simulink model "UR5e_Unreal_Checkpoint"  (R2025b)
settings: Solver=FixedStepDiscrete  StartTime=0.0  StopTime=stopTimeUE  FixedStep=0.02  RelTol=1e-3
values from neighbouring files (symbols this model uses):
  qUE = qMotion(1,:)    [UR5e_Prepare_Project.m]    (also in UR5e_UE_Scene.m)
undefined symbols (not defined in the file or in its folder): Actor, UR5e_Glue_Bead
libraries: sim3dlib x2, robotsim3dlib x1
settings Model: Creator=Lenovo  LastModifiedBy=Lenovo

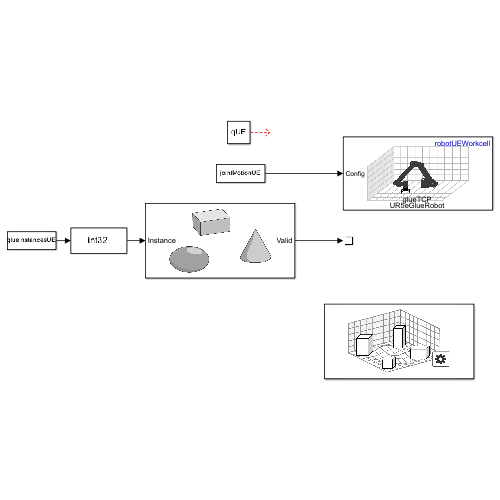
[thumbnail: Simulink's stored preview of the top-level diagram]
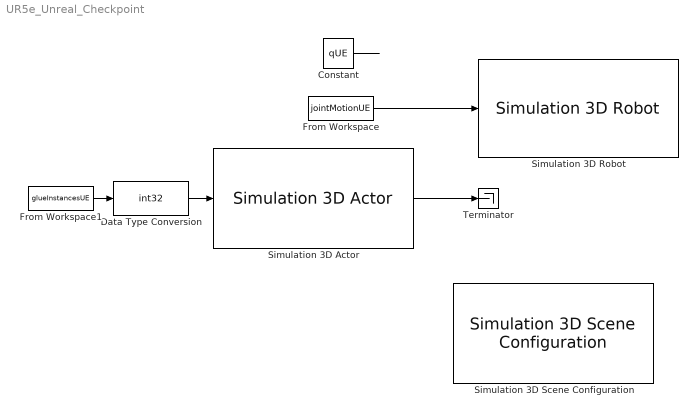
== system UR5e_Unreal_Checkpoint ==
  Constant : Constant  Value=qUE
  Data Type Conversion : DataTypeConversion  OutDataTypeStr=int32  SaturateOnIntegerOverflow=off  RndMeth=Floor
  From Workspace : FromWorkspace  VariableName=jointMotionUE  SampleTime=0.02  OutputAfterFinalValue=Holding final value
  From Workspace1 : FromWorkspace  VariableName=glueInstancesUE  SampleTime=0.02  Interpolate=off  OutputAfterFinalValue=Holding final value
  Simulation 3D Actor : sim3dlib/Simulation 3D Actor  Priority=-1  ActorName=GlueBead  ParentName=Scene Origin  Operation=Create at step  InitScriptText=UR5e_Glue_Bead('create', Actor);  SampleTime=-1  Translation=[0 0 0]  Rotation=[0 0 0]  Scale=[1 1 1]  aMode=5  ActorTag=Sim3dActor1  ActorType=Sim3dActor  ID=1
  Simulation 3D Robot : robotsim3dlib/Simulation 3D Robot  actorInputType=RigidBodyTree Object  RigidBodyTree=robotUEWorkcell  ActorName=UR5eGlueRobot  existActorChekBox=off  initialTrans=[0 0 0]  initialRot=[0 0 0]  initialConfig=qUE  EndEffector=glueTCP  eeOffsetInpChekBox=off  eeTargetTrans=[0 0 0]  eeTargetRot=[0 0 0]  enableRegionGraspChekBox=off  regionGraspInpChekBox=off  eeTargTransDiff=[0.2 0.2 0.2]  eeTargRotDiff=[0 0 0]  enableVisualVisualization=on  enableCollisionVisualization=off  collisionGeomColor=[0 1 0]  collisionGeomTransp=0.1  inpConfEnbVal=on  inpGraspEnbVal=off  inpTransEnbVal=off  outConfEnbVal=off  outGraspEnbVal=off  outTransEnbVal=off  SampleTime=0.02  ActorType=SimulinkVehicle  ID=C  aMode=6  ActorTag=UR5eGlueRobot  Mesh=RigidBodyTree
  Simulation 3D Scene Configuration : sim3dlib/Simulation 3D Scene Configuration  Priority=0  ProjectFormat=Default Scenes  SceneDesc=Empty scene  ProjectName=C:\Program Files\MATLAB\R2025b\toolbox\shared\sim3d_projects\automotive_project_windows\UE\WindowsNoEditor\VehicleSimulation.exe  ScenePath=/Game/Maps/EmptyScene  EnableOpenDRIVE=off  vehTagList={'<empty>';'Custom';'Scene Origin';'UR5eGlueRobot'}  vehTag=Scene Origin  AttachedCameraRelativeTranslation=[0 0 0]  FreeCameraDefaultInitialTranslation=[-6, 0, 2]  AttachedCameraRelativeRotation=[0 0 0]  FreeCameraDefaultInitialRotation=[0, -15, 0]  ViewpointName=Custom  FreeCameraInitialTranslation=[0 0 0]  ViewpointTranslation=[0 0 0]  FreeCameraInitialRotation=[0 0 0]  ViewpointRotation=[0 0 0]  OpVisEn=off  Ts=0.02  EnableWindow=on  EnableRemoteAccess=off  EnableWeather=off  SunAzimuth=90  SunAltitude=40.0  EnableGeospatialSun=off  Latitude=0  Longitude=0  Date=2023-01-01  Time=10:30:00  GeoTimeZone=-5.0  SunDaylightSaving=off  wind=1  clouds=10  EnableVolumetricClouds=off  CloudCoverage=0  CloudAltitude=6  fog=0  rain=0  RaindropsEffect=off  SnowDensity=0  EnableGeospatial=off  TilesetSource=Earth terrain  UseTrueOrigin=off  OriginHeight=200  OriginLatitude=40.744652  OriginLongitude=-73.988864  MapStyle=Aerial  AdditionalAssetIDs=[]  UseAdvancedSunSky=off  SolarTime=11  TimeZone=-5  Day=21  Month=9  Year=2022  UseDaylightSavingTime=on  DSTStartDay=10  DSTStartMonth=3  DSTEndDay=3  DSTEndMonth=11  DSTSwitchHour=2  sensorTag=MainCamera1  sensorId=1  sensorName=MainCamera1  mountLoc=Origin  offsetFlag=off  tmountOffset=[0, 0, 0]  rmountOffset=[0, 0, 0]  HorizontalResolution=1280  VerticalResolution=720  HorizontalFOV=60  mountPoint=[0 0 0]  mountOrientation=[0 0 0]  aMode=6  ID=1  GeoTrigger=Inactive  ViewNameList={'Custom'}  ViewTranslationList={'[0 0 0]'}  ViewRotationList={'[0 0 0]'}
      settings: LibrarySourceBlock=robotsim3dlib/Simulation 3D Scene Configuration
  Terminator : Terminator
  wires:
  Constant/1 -> ?
  From Workspace/1 -> Simulation 3D Robot/1
  From Workspace1/1 -> Data Type Conversion/1
  Data Type Conversion/1 -> Simulation 3D Actor/1
  Simulation 3D Actor/1 -> Terminator/1
